simulink model "dcmotor_cascade"  (R2024b)
settings: Solver=ode45  StartTime=0.0  StopTime=2  MaxStep=1e-4  RelTol=1e-6
InitFcn:
  | cascade_params; apply_scenario;
undefined symbols (not defined in the file): ctrl, motor, scn
libraries: slpidlib x2
Description:
  | v0.2 cascade DC motor drive: speed PI (1 kHz) -> current PI (10 kHz, 5 A limit).
settings Model: Creator=HP PC  LastModifiedBy=HP PC

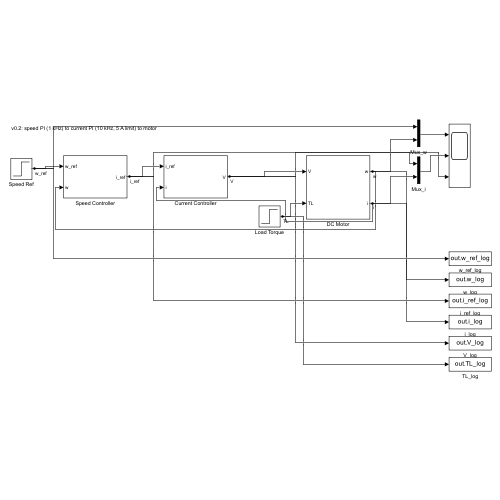
[thumbnail: Simulink's stored preview of the top-level diagram]
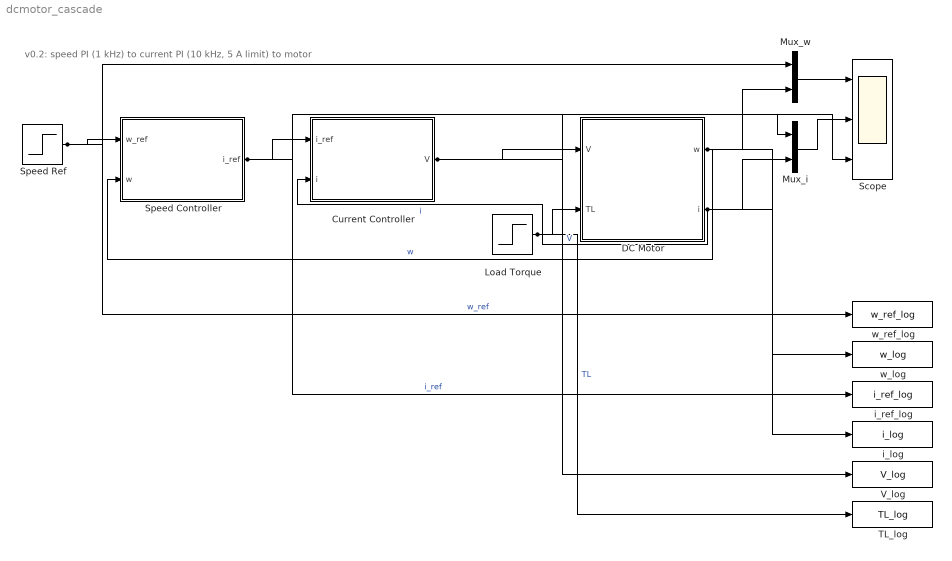
== system dcmotor_cascade ==
  note: v0.2: speed PI (1 kHz) to current PI (10 kHz, 5 A limit) to motor
  Current Controller : Subsystem
  DC Motor : Subsystem
  Load Torque : Step  Time=scn.t_load  After=scn.TL  SampleTime=0
  Mux_i : Mux  Inputs=2
  Mux_w : Mux  Inputs=2
  Scope : Scope  NumInputPorts=3
  Speed Controller : Subsystem
  Speed Ref : Step  Time=scn.t_ref  After=scn.w_ref  SampleTime=0
  TL_log : ToWorkspace  VariableName=TL_log  SaveFormat=Timeseries  SampleTime=-1
  V_log : ToWorkspace  VariableName=V_log  SaveFormat=Timeseries  SampleTime=-1
  i_log : ToWorkspace  VariableName=i_log  SaveFormat=Timeseries  SampleTime=-1
  i_ref_log : ToWorkspace  VariableName=i_ref_log  SaveFormat=Timeseries  SampleTime=-1
  w_log : ToWorkspace  VariableName=w_log  SaveFormat=Timeseries  SampleTime=-1
  w_ref_log : ToWorkspace  VariableName=w_ref_log  SaveFormat=Timeseries  SampleTime=-1
  wires:
  Speed Ref/1 -> Speed Controller/1(w_ref), Mux_w/1, w_ref_log/1  "w_ref"
  Speed Controller/1(i_ref) -> Current Controller/1(i_ref), Mux_i/1, i_ref_log/1  "i_ref"
  Current Controller/1(V) -> DC Motor/1(V), Scope/3, V_log/1  "V"
  Load Torque/1 -> DC Motor/2(TL), TL_log/1  "TL"
  DC Motor/1(w) -> Speed Controller/2(w), Mux_w/2, w_log/1  "w"
  DC Motor/2(i) -> Current Controller/2(i), Mux_i/2, i_log/1  "i"
  Mux_w/1 -> Scope/1
  Mux_i/1 -> Scope/2

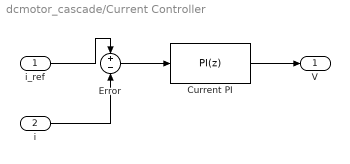
== system dcmotor_cascade/Current Controller ==
  i_ref : Inport
  i : Inport  Port=2
  Current PI : slpidlib/PID Controller  Controller=PI  Form=Parallel  TimeDomain=Discrete-time  UseExternalTs=off  SampleTime=ctrl.Ts_i  IntegratorMethod=Forward Euler  FilterMethod=Forward Euler  ControllerParametersSource=internal  P=ctrl.Kp_i  I=ctrl.Ki_i  UseKiTs=off  D=0  UseExternalDerivativeSource=off  N=100  UseFilter=on  TunerSelectOption=Transfer Function Based (PID Tuner App)  InitialConditionSource=internal  InitialConditionForIntegrator=0  InitialConditionForFilter=0  DifferentiatorICPrevScaledInput=0  ExternalReset=none  TrackingMode=off  Kt=1  LimitOutput=on  SatLimitsSource=internal  UpperSaturationLimit=ctrl.Vmax  LowerSaturationLimit=-ctrl.Vmax  LinearizeAsGain=on  AntiWindupMode=clamping  Kb=1  LimitIntegrator=off  UpperIntegratorSaturationLimit=inf  LowerIntegratorSaturationLimit=-inf  POutMin=[]  POutMax=[]  IOutMin=[]  IOutMax=[]  DOutMin=[]  DOutMax=[]  NOutMin=[]  NOutMax=[]  SumOutMin=[]  SumOutMax=[]  SaturationOutMin=[]  SaturationOutMax=[]  PParamMin=[]  PParamMax=[]  IParamMin=[]  IParamMax=[]  DParamMin=[]  DParamMax=[]  NParamMin=[]  NParamMax=[]  KbParamMin=[]  KbParamMax=[]  KtParamMin=[]  KtParamMax=[]  KbOutMin=[]  KbOutMax=[]  KtOutMin=[]  KtOutMax=[]  IntegratorOutMin=[]  IntegratorOutMax=[]  FilterOutMin=[]  FilterOutMax=[]  SumI1OutMin=[]  SumI1OutMax=[]  SumI2OutMin=[]  SumI2OutMax=[]  SumI3OutMin=[]  SumI3OutMax=[]  SumI4OutMin=[]  SumI4OutMax=[]  SumDOutMin=[]  SumDOutMax=[]  DifferentiatorOutMin=[]  DifferentiatorOutMax=[]  FilterDiffOutCoefMin=[]  FilterDiffOutCoefMax=[]  ReciprocalOutMin=[]  ReciprocalOutMax=[]  SumDenOutMin=[]  SumDenOutMax=[]  SumNumOutMin=[]  SumNumOutMax=[]  DivideOutMin=[]  DivideOutMax=[]  UdiffTsProdOutMin=[]  UdiffTsProdOutMax=[]  NTsProdOutMin=[]  NTsProdOutMax=[]  UintegralTsProdOutMin=[]  UintegralTsProdOutMax=[]  UngainTsProdOutMin=[]  UngainTsProdOutMax=[]  ClampingZeroOutDataTypeStr=Inherit: Inherit via back propagation  ClampingZeroOutMin=[]  ClampingZeroOutMax=[]  FilterDenConstantOutDataTypeStr=Inherit: Inherit via back propagation  FilterDenConstantOutMin=[]  FilterDenConstantOutMax=[]  PCopyOutDataTypeStr=Inherit: Inherit via back propagation  PCopyOutMin=[]  PCopyOutMax=[]  NCopyOutDataTypeStr=Inherit: Inherit via back propagation  NCopyOutMin=[]  NCopyOutMax=[]  IntegratorContinuousStateAttributes=''  IntegratorStateMustResolveToSignalObject=off  IntegratorRTWStateStorageClass=Auto  FilterContinuousStateAttributes=''  FilterStateMustResolveToSignalObject=off  FilterRTWStateStorageClass=Auto  ParallelPVariant=InternalParameters  IdealPVariant=Disabled  IVariant=InternalParameters  DVariant=Disabled  IntegratorVariant=Discrete  SatVariant=Enabled  AWVariant=DiscClampingParallel  PCopyVariant=Disabled  TRVariant=Disabled  FdbkBlocksVariant=Forward  IdealPFdbkVariant=Disabled  SatFdbkVariant=Disabled  DerivativeFilterVariant=Disabled  NVariant=Disabled  NCopyVariant=Disabled_SignalSpec  FilterICVariant=Disabled  IntegratorICVariant=InternalICs  ExternalResetVariant=Disabled  TRSumVariant=Passthrough  SumFdbkVariant=Disabled  SumVariant=Sum_PI  TsampFilterVariant=InternalTs  TsampNgainVariant=Passthrough  TsampIntegralVariant=Disabled_SignalSpec  ExternalSaturationOutDataTypeStr=Inherit: Same as second input  DerivativeSourceVariant=Disabled  PreIntVariant=InternalPreInt
  Error : Sum  Inputs=+-
  V : Outport
  wires:
  i_ref/1 -> Error/1
  i/1 -> Error/2
  Error/1 -> Current PI/1
  Current PI/1 -> V/1

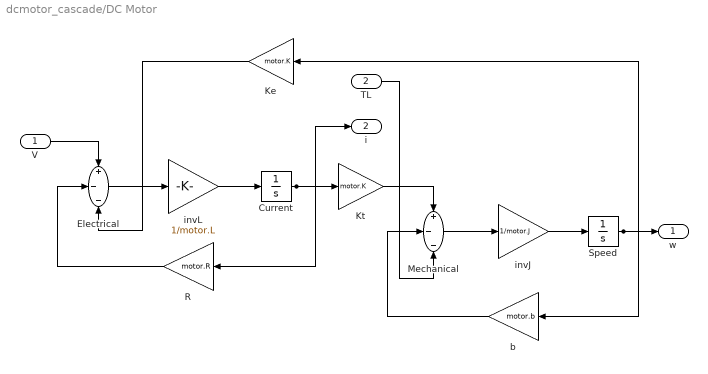
== system dcmotor_cascade/DC Motor ==
  V : Inport
  TL : Inport  Port=2
  Current : Integrator  InitialCondition=motor.i0
  Electrical : Sum  Inputs=+--
  Ke : Gain  Gain=motor.K
  Kt : Gain  Gain=motor.K
  Mechanical : Sum  Inputs=+--
  R : Gain  Gain=motor.R
  Speed : Integrator  InitialCondition=motor.w0
  b : Gain  Gain=motor.b
  invJ : Gain  Gain=1/motor.J
  invL : Gain  Gain=1/motor.L
  w : Outport
  i : Outport  Port=2
  wires:
  V/1 -> Electrical/1
  R/1 -> Electrical/2
  b/1 -> Mechanical/2
  TL/1 -> Mechanical/3
  Electrical/1 -> invL/1
  invL/1 -> Current/1
  Ke/1 -> Electrical/3
  Kt/1 -> Mechanical/1
  Current/1 -> R/1, Kt/1, i/1
  Mechanical/1 -> invJ/1
  invJ/1 -> Speed/1
  Speed/1 -> b/1, Ke/1, w/1

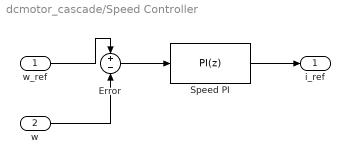
== system dcmotor_cascade/Speed Controller ==
  w_ref : Inport
  w : Inport  Port=2
  Error : Sum  Inputs=+-
  Speed PI : slpidlib/PID Controller  Controller=PI  Form=Parallel  TimeDomain=Discrete-time  UseExternalTs=off  SampleTime=ctrl.Ts_w  IntegratorMethod=Forward Euler  FilterMethod=Forward Euler  ControllerParametersSource=internal  P=ctrl.Kp_w  I=ctrl.Ki_w  UseKiTs=off  D=0  UseExternalDerivativeSource=off  N=100  UseFilter=on  TunerSelectOption=Transfer Function Based (PID Tuner App)  InitialConditionSource=internal  InitialConditionForIntegrator=0  InitialConditionForFilter=0  DifferentiatorICPrevScaledInput=0  ExternalReset=none  TrackingMode=off  Kt=1  LimitOutput=on  SatLimitsSource=internal  UpperSaturationLimit=ctrl.Imax  LowerSaturationLimit=-ctrl.Imax  LinearizeAsGain=on  AntiWindupMode=clamping  Kb=1  LimitIntegrator=off  UpperIntegratorSaturationLimit=inf  LowerIntegratorSaturationLimit=-inf  POutMin=[]  POutMax=[]  IOutMin=[]  IOutMax=[]  DOutMin=[]  DOutMax=[]  NOutMin=[]  NOutMax=[]  SumOutMin=[]  SumOutMax=[]  SaturationOutMin=[]  SaturationOutMax=[]  PParamMin=[]  PParamMax=[]  IParamMin=[]  IParamMax=[]  DParamMin=[]  DParamMax=[]  NParamMin=[]  NParamMax=[]  KbParamMin=[]  KbParamMax=[]  KtParamMin=[]  KtParamMax=[]  KbOutMin=[]  KbOutMax=[]  KtOutMin=[]  KtOutMax=[]  IntegratorOutMin=[]  IntegratorOutMax=[]  FilterOutMin=[]  FilterOutMax=[]  SumI1OutMin=[]  SumI1OutMax=[]  SumI2OutMin=[]  SumI2OutMax=[]  SumI3OutMin=[]  SumI3OutMax=[]  SumI4OutMin=[]  SumI4OutMax=[]  SumDOutMin=[]  SumDOutMax=[]  DifferentiatorOutMin=[]  DifferentiatorOutMax=[]  FilterDiffOutCoefMin=[]  FilterDiffOutCoefMax=[]  ReciprocalOutMin=[]  ReciprocalOutMax=[]  SumDenOutMin=[]  SumDenOutMax=[]  SumNumOutMin=[]  SumNumOutMax=[]  DivideOutMin=[]  DivideOutMax=[]  UdiffTsProdOutMin=[]  UdiffTsProdOutMax=[]  NTsProdOutMin=[]  NTsProdOutMax=[]  UintegralTsProdOutMin=[]  UintegralTsProdOutMax=[]  UngainTsProdOutMin=[]  UngainTsProdOutMax=[]  ClampingZeroOutDataTypeStr=Inherit: Inherit via back propagation  ClampingZeroOutMin=[]  ClampingZeroOutMax=[]  FilterDenConstantOutDataTypeStr=Inherit: Inherit via back propagation  FilterDenConstantOutMin=[]  FilterDenConstantOutMax=[]  PCopyOutDataTypeStr=Inherit: Inherit via back propagation  PCopyOutMin=[]  PCopyOutMax=[]  NCopyOutDataTypeStr=Inherit: Inherit via back propagation  NCopyOutMin=[]  NCopyOutMax=[]  IntegratorContinuousStateAttributes=''  IntegratorStateMustResolveToSignalObject=off  IntegratorRTWStateStorageClass=Auto  FilterContinuousStateAttributes=''  FilterStateMustResolveToSignalObject=off  FilterRTWStateStorageClass=Auto  ParallelPVariant=InternalParameters  IdealPVariant=Disabled  IVariant=InternalParameters  DVariant=Disabled  IntegratorVariant=Discrete  SatVariant=Enabled  AWVariant=DiscClampingParallel  PCopyVariant=Disabled  TRVariant=Disabled  FdbkBlocksVariant=Forward  IdealPFdbkVariant=Disabled  SatFdbkVariant=Disabled  DerivativeFilterVariant=Disabled  NVariant=Disabled  NCopyVariant=Disabled_SignalSpec  FilterICVariant=Disabled  IntegratorICVariant=InternalICs  ExternalResetVariant=Disabled  TRSumVariant=Passthrough  SumFdbkVariant=Disabled  SumVariant=Sum_PI  TsampFilterVariant=InternalTs  TsampNgainVariant=Passthrough  TsampIntegralVariant=Disabled_SignalSpec  ExternalSaturationOutDataTypeStr=Inherit: Same as second input  DerivativeSourceVariant=Disabled  PreIntVariant=InternalPreInt
  i_ref : Outport
  wires:
  w_ref/1 -> Error/1
  w/1 -> Error/2
  Error/1 -> Speed PI/1
  Speed PI/1 -> i_ref/1
